simulink model "pwm"  (R2026b)
settings: Solver=FixedStepAuto  StopTime=inf  EnableMultiTasking=on
libraries: stm32f4xxblockslib x3
settings Model: STM32="{\"PWMOutput\":{\"ID\":\"2\"},\"DigitalPortWrite\":[{\"ID\":\"10\"},{\"ID\":\"11\"}]}"  Creator=sanka  LastModifiedBy=sanka
settings OptimizationCC: DifferentSizesBufferReuse=on  EfficientTunableParamExpr=on  EnhancedBackFolding=on  MaxStackSize=512  OptimizationCustomize=off  OptimizeBlockOrder=speed  PassReuseOutputArgsAs=Individual arguments  RemoveInternalMemoryZeroInit=on  RemoveRootLevelIOMemoryZeroInit=on
settings DebuggingCC: ParameterTunabilityLossMsg=error
settings HardwareCC: ProdHWDeviceType=ARM Compatible->ARM Cortex-M  ProdLargestAtomicFloat=Double  ProdLargestAtomicInteger=Long  ProdLongLongMode=on
settings SFSimCC: MATLABDynamicMemAlloc=off
settings RTWCC: BuildConfiguration=Faster Runs  Description=Embedded Coder  HardwareBoard=STM32F4xx Based  SystemTargetFile=ert.tlc  TLCOptions=-aInlineSetEventsForThisBaseRateFcn=TLC_FALSE -aSuppressMultiTaskScheduler=TLC_FALSE -aRateBasedStepFcn=1  TemplateMakefile=ert_default_tmf  Toolchain=GNU Tools for STM32
settings CodeAppCC: ForceParamTrailComments=on  IgnoreCustomStorageClasses=off  InsertBlockDesc=on  OperatorAnnotations=on  SFDataObjDesc=on  SimulinkDataObjDesc=on
settings ERTTargetCC: CodeReplacementLibrary=ARM Cortex-M  CombineSignalStateStructs=on  ExtModeIntrfLevel=Level2 - Open  ExtModeMexFile=ext_xcp  ExtModeStaticAlloc=on

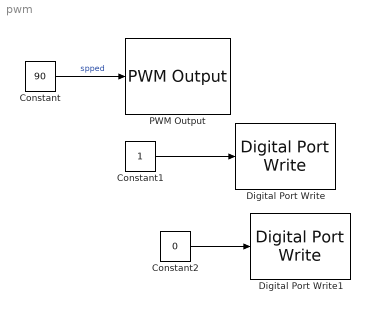
== system pwm ==
  Constant : Constant  Value=90
  Constant1 : Constant
  Constant2 : Constant  Value=0
  Digital Port Write : stm32f4xxblockslib/Digital Port Write  PortName=GPIOA  PinNumber=[0]  ReadOperation=off  IOAsArray=on  EnableSimPort=off  hoistedMaskSrc=ECSoC/ECSimCodegen/Digital Port Write
  Digital Port Write1 : stm32f4xxblockslib/Digital Port Write  PortName=GPIOA  PinNumber=[1]  ReadOperation=off  IOAsArray=on  EnableSimPort=off  hoistedMaskSrc=ECSoC/ECSimCodegen/Digital Port Write
  PWM Output : stm32f4xxblockslib/PWM Output  ProcessorFamily=STM32F4  TimerModule=TIM1  DutycycleUnits=Percentage  EnableChannel1=on  EnableCaptureCompare1Input=off  EnableCaptureCompare1ComplementaryInput=off  EnableOutputCompare1ModeInput=off  EnableChannel2=off  EnableCaptureCompare2Input=off  EnableCaptureCompare2ComplementaryInput=off  EnableOutputCompare2ModeInput=off  EnableChannel3=off  EnableCaptureCompare3Input=off  EnableCaptureCompare3ComplementaryInput=off  EnableOutputCompare3ModeInput=off  EnableChannel4=off  EnableCaptureCompare4Input=off  EnableCaptureCompare4ComplementaryInput=off  EnableOutputCompare4ModeInput=off  EnableChannel5=off  EnableCaptureCompare5Input=off  EnableOutputCompare5ModeInput=off  EnableChannel6=off  EnableCaptureCompare6Input=off  EnableOutputCompare6ModeInput=off  EnableCounterInput=off  EnableMainOutputInput=off  EnableFrequencyInput=off  SetRCAfterCE=off  OutputDirection=off  OutputMainOutputEnableStatus=off  SampleTime=0.1  EnableSimPort=off  EnableUpdateEvent=off  EnableCaptureCompare1Event=off  EnableCaptureCompare2Event=off  EnableCaptureCompare3Event=off  EnableCaptureCompare4Event=off  EnableTriggerEvent=off  EnableBreakEvent=off  EnableBreakEvent2=off  hoistedMaskSrc=ECSoC/ECSimCodegen/PWM Output
  wires:
  Constant/1 -> PWM Output/1  "spped"
  Constant1/1 -> Digital Port Write/1
  Constant2/1 -> Digital Port Write1/1
